simulink model "High_speed_sim"  (R2016a)
settings: Solver=VariableStepAuto  StartTime=0.0  StopTime=2  RelTol=1e-3
values from neighbouring files (symbols this model uses):
  DL = 2*psi*sqrt(KL*JL)    [High_speed.m]
  JL = NL*(Ng^2)*Jm    (= 0.00027)    [High_speed.m]
  Jm = 0.000054    (= 5.4e-05)    [High_speed.m]
  KL = (wL^2)*JL    (= 2.3958828)    [High_speed.m]
  Kp = cp*wL    (= 22.608)    [High_speed.m]
  Kvg = (Jm+JL/Ng^2)*Kv    (= 0.025027056)    [High_speed.m]
  Ng = 1    [High_speed.m]
libraries: simulink x1
settings Model: Creator=DELL  LastModifiedBy=DELL

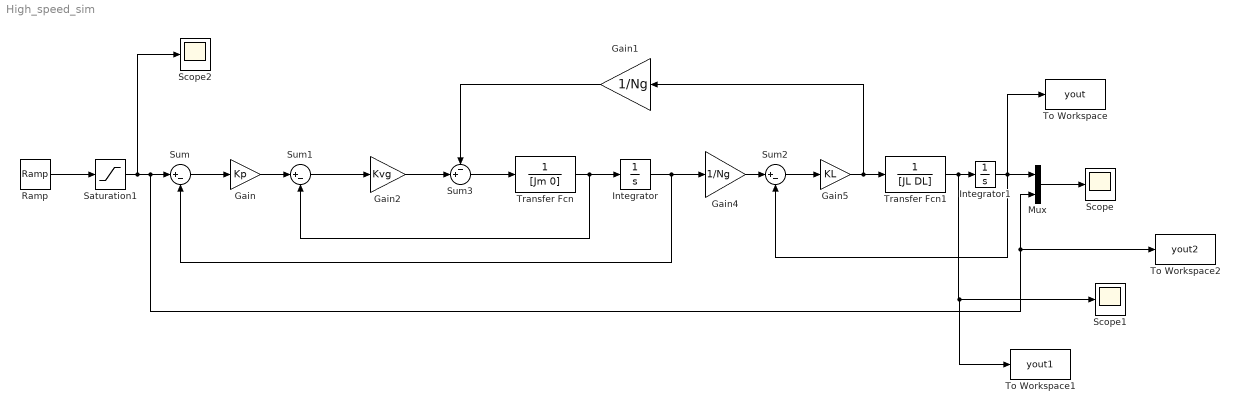
== system High_speed_sim ==
  Gain : Gain  Gain=Kp
  Gain1 : Gain  Gain=1/Ng
  Gain2 : Gain  Gain=Kvg
  Gain4 : Gain  Gain=1/Ng
  Gain5 : Gain  Gain=KL
  Integrator : Integrator
  Integrator1 : Integrator
  Mux : Mux  Inputs=2
  Ramp : simulink/Sources/Ramp  slope=50  start=0  X0=0
  Saturation1 : Saturate  UpperLimit=10  LowerLimit=0
  Scope : Scope
  Scope1 : Scope
  Scope2 : Scope
  Sum : Sum  Inputs=|+-
  Sum1 : Sum  Inputs=|+-
  Sum2 : Sum  Inputs=|+-
  Sum3 : Sum  Inputs=-+|
  To Workspace : ToWorkspace  VariableName=yout  SaveFormat=Timeseries  SampleTime=-1
  To Workspace1 : ToWorkspace  VariableName=yout1  SaveFormat=Timeseries  SampleTime=-1
  To Workspace2 : ToWorkspace  VariableName=yout2  SaveFormat=Timeseries  SampleTime=-1
  Transfer Fcn : TransferFcn  Denominator=[Jm 0]
  Transfer Fcn1 : TransferFcn  Denominator=[JL DL]
  wires:
  Transfer Fcn1/1 -> To Workspace1/1, Scope1/1, Integrator1/1
  Sum1/1 -> Gain2/1
  Integrator/1 -> Sum/2, Gain4/1
  Gain4/1 -> Sum2/1
  Transfer Fcn/1 -> Integrator/1, Sum1/2
  Gain2/1 -> Sum3/2
  Sum3/1 -> Transfer Fcn/1
  Gain1/1 -> Sum3/1
  Sum/1 -> Gain/1
  Gain/1 -> Sum1/1
  Gain5/1 -> Gain1/1, Transfer Fcn1/1
  Ramp/1 -> Saturation1/1
  Mux/1 -> Scope/1
  Sum2/1 -> Gain5/1
  Integrator1/1 -> Sum2/2, Mux/1, To Workspace/1
  Saturation1/1 -> Scope2/1, Sum/1, To Workspace2/1, Mux/2
